simulink model "sm_car_"  (R2026b)
settings: Solver=ode23t  StopTime=100  MaxStep=0.4  AbsTol=1e-3  EnableMultiTasking=on
PreLoadFcn:
  | % Due to usability issue in Repeating Sequence block
  | warning('off','Simulink:Masking:Invalid');
  | 
  | % Eliminate unnecessary warnings in inactive variants
  | % Warnings generated only if you click through inactive variant
  | warning('off','MATLAB:nonExistentField');
  | warning('off','Simulink:Parameters:BlkParamUndefined');
PostLoadFcn:
  | set_param([bdroot '/Vehicle'],'popup_trailer','Off')
  | warning('off','sm:sli:setup:compile:LocalSolverNotSupported')
  | %sm_car_config_maneuver(bdroot,'WOT Braking');
  | sm_car_config_vehicle(bdroot,'false');
  | sm_car_config_logging(bdroot);
InitFcn:
  | sm_car_config_camera;
  | Vehicle = sm_car_vehcfg_checkConfig(Vehicle);
  | sm_car_check_tire_model(bdroot);
StartFcn:
  | tic;
StopFcn:
  | Elapsed_Sim_Time = toc;
  | % disp(['Elapsed Sim Time = ' num2str(Elapsed_Sim_Time)]);
undefined symbols (not defined in the file or in its folder): acc_theta, accel_ramp_rate, Axle1D, AxleIn, Camera, Control, Driver, Init, Maneuver, Pedal, Scene, ShaftL1, ShaftL2, ShaftR1, ShaftR2, Visual, X, xy_data_car_side, Y, Z
libraries: sm_lib x290, fl_lib x171, nesl_utility x144, simulink x60, simulink_extras x14, sdl_lib x14, SimscapeFluids_lib x7, Damper_Element x4, Tire_1x2x x4, ee_lib x3, Scene_Utilities x3, sharedTrackingLibrary x2
(part 17 of 22)

== system sm_car_/World/Scene/CRG Hockenheim F/Finish Line/R5 ==
  Square LL : sm_lib/Body Elements/Brick Solid  BrickDimensions=square_lwh  BrickDimensionsUnits=m  ExportEntireGeometry=off  InertiaType=CalculateFromGeometry  BasedOnType=Density  Density=1000  DensityUnits=kg/m^3  Mass=1  MassUnits=kg  CenterOfMass=[0 0 0]  CenterOfMassUnits=m  MomentsOfInertia=[1 1 1]  MomentsOfInertiaUnits=kg*m^2  ProductsOfInertia=[0 0 0]  ProductsOfInertiaUnits=kg*m^2  GraphicType=FromGeometry  MarkerShape=Sphere  MarkerSize=10  GraphicVisPropType=SimpleVisualProperties  GraphicDiffuseColor=[0.0 0.0 0.0]  GraphicOpacity=1.0  GraphicSpecularColor=[0.5 0.5 0.5 1.0]  GraphicAmbientColor=[0.15 0.15 0.15 1.0]  GraphicEmissiveColor=[0.0 0.0 0.0 1.0]  GraphicShininess=75  DoExposeReferenceFrame=off  SerializedFrames=<Frames><Frame><Id>Frame1</Id><Value><Name>BL</Name><Origin><Source>GeometricFeature</Source><FeatureName>+y -z curve</FeatureName></Origin><PrimaryAxis><DefinedDirection>+Z</DefinedDirection><Source>ReferenceFrame</Source><SourceDirection>+Z</SourceDirection><FeatureName></FeatureName></PrimaryAxis><SecondaryAxis><DefinedDirection>+X</DefinedDirection><Source>ReferenceFrame</Source><SourceDirection>+X</SourceDirection><FeatureName></FeatureName></SecondaryAxis></Value></Frame><Frame><Id>Frame2</Id><Value><Name>TL</Name><Origin><Source>GeometricFeature</Source><FeatureName>+x +y +z point</FeatureName></Origin><PrimaryAxis><DefinedDirection>+Z</DefinedDirection><Source>ReferenceFrame</Source><SourceDirection>+Z</SourceDirection><FeatureName></FeatureName></PrimaryAxis><SecondaryAxis><DefinedDirection>+X</DefinedDirection><Source>ReferenceFrame</Source><SourceDirection>+X</SourceDirection><FeatureName></FeatureName></SecondaryAxis></Value></Frame><Frame><Id>Frame3</Id><Value><Name>BR</Name><Origin><Source>GeometricFeature</Source><FeatureName>-y -z curve</FeatureName></Origin><PrimaryAxis><DefinedDirection>+Z</DefinedDirection><Source>ReferenceFrame</Source><SourceDirection>+Z</SourceDirection><FeatureName></FeatureName></PrimaryAxis><SecondaryAxis><DefinedDirection>+X</DefinedDirection><Source>ReferenceFrame</Source><SourceDirection>+X</SourceDirection><FeatureName></FeatureName></SecondaryAxis></Value></Frame></Frames>
  Square LR : sm_lib/Body Elements/Brick Solid  BrickDimensions=square_lwh  BrickDimensionsUnits=m  ExportEntireGeometry=off  InertiaType=CalculateFromGeometry  BasedOnType=Density  Density=1000  DensityUnits=kg/m^3  Mass=1  MassUnits=kg  CenterOfMass=[0 0 0]  CenterOfMassUnits=m  MomentsOfInertia=[1 1 1]  MomentsOfInertiaUnits=kg*m^2  ProductsOfInertia=[0 0 0]  ProductsOfInertiaUnits=kg*m^2  GraphicType=FromGeometry  MarkerShape=Sphere  MarkerSize=10  GraphicVisPropType=SimpleVisualProperties  GraphicDiffuseColor=[1.0 1.0 1.0]  GraphicOpacity=1.0  GraphicSpecularColor=[0.5 0.5 0.5 1.0]  GraphicAmbientColor=[0.15 0.15 0.15 1.0]  GraphicEmissiveColor=[0.0 0.0 0.0 1.0]  GraphicShininess=75  DoExposeReferenceFrame=off  SerializedFrames=<Frames><Frame><Id>Frame1</Id><Value><Name>BL</Name><Origin><Source>GeometricFeature</Source><FeatureName>+y -z curve</FeatureName></Origin><PrimaryAxis><DefinedDirection>+Z</DefinedDirection><Source>ReferenceFrame</Source><SourceDirection>+Z</SourceDirection><FeatureName></FeatureName></PrimaryAxis><SecondaryAxis><DefinedDirection>+X</DefinedDirection><Source>ReferenceFrame</Source><SourceDirection>+X</SourceDirection><FeatureName></FeatureName></SecondaryAxis></Value></Frame><Frame><Id>Frame2</Id><Value><Name>TL</Name><Origin><Source>GeometricFeature</Source><FeatureName>+x +y +z point</FeatureName></Origin><PrimaryAxis><DefinedDirection>+Z</DefinedDirection><Source>ReferenceFrame</Source><SourceDirection>+Z</SourceDirection><FeatureName></FeatureName></PrimaryAxis><SecondaryAxis><DefinedDirection>+X</DefinedDirection><Source>ReferenceFrame</Source><SourceDirection>+X</SourceDirection><FeatureName></FeatureName></SecondaryAxis></Value></Frame><Frame><Id>Frame3</Id><Value><Name>BR</Name><Origin><Source>GeometricFeature</Source><FeatureName>-y -z curve</FeatureName></Origin><PrimaryAxis><DefinedDirection>+Z</DefinedDirection><Source>ReferenceFrame</Source><SourceDirection>+Z</SourceDirection><FeatureName></FeatureName></PrimaryAxis><SecondaryAxis><DefinedDirection>+X</DefinedDirection><Source>ReferenceFrame</Source><SourceDirection>+X</SourceDirection><FeatureName></FeatureName></SecondaryAxis></Value></Frame></Frames>
  Square UL : sm_lib/Body Elements/Brick Solid  BrickDimensions=square_lwh  BrickDimensionsUnits=m  ExportEntireGeometry=off  InertiaType=CalculateFromGeometry  BasedOnType=Density  Density=1000  DensityUnits=kg/m^3  Mass=1  MassUnits=kg  CenterOfMass=[0 0 0]  CenterOfMassUnits=m  MomentsOfInertia=[1 1 1]  MomentsOfInertiaUnits=kg*m^2  ProductsOfInertia=[0 0 0]  ProductsOfInertiaUnits=kg*m^2  GraphicType=FromGeometry  MarkerShape=Sphere  MarkerSize=10  GraphicVisPropType=SimpleVisualProperties  GraphicDiffuseColor=[1.0 1.0 1.0]  GraphicOpacity=1.0  GraphicSpecularColor=[0.5 0.5 0.5 1.0]  GraphicAmbientColor=[0.15 0.15 0.15 1.0]  GraphicEmissiveColor=[0.0 0.0 0.0 1.0]  GraphicShininess=75  DoExposeReferenceFrame=off  SerializedFrames=<Frames><Frame><Id>Frame1</Id><Value><Name>BL</Name><Origin><Source>GeometricFeature</Source><FeatureName>+y -z curve</FeatureName></Origin><PrimaryAxis><DefinedDirection>+Z</DefinedDirection><Source>ReferenceFrame</Source><SourceDirection>+Z</SourceDirection><FeatureName></FeatureName></PrimaryAxis><SecondaryAxis><DefinedDirection>+X</DefinedDirection><Source>ReferenceFrame</Source><SourceDirection>+X</SourceDirection><FeatureName></FeatureName></SecondaryAxis></Value></Frame><Frame><Id>Frame2</Id><Value><Name>TL</Name><Origin><Source>GeometricFeature</Source><FeatureName>+x +y +z point</FeatureName></Origin><PrimaryAxis><DefinedDirection>+Z</DefinedDirection><Source>ReferenceFrame</Source><SourceDirection>+Z</SourceDirection><FeatureName></FeatureName></PrimaryAxis><SecondaryAxis><DefinedDirection>+X</DefinedDirection><Source>ReferenceFrame</Source><SourceDirection>+X</SourceDirection><FeatureName></FeatureName></SecondaryAxis></Value></Frame><Frame><Id>Frame3</Id><Value><Name>BR</Name><Origin><Source>GeometricFeature</Source><FeatureName>-y -z curve</FeatureName></Origin><PrimaryAxis><DefinedDirection>+Z</DefinedDirection><Source>ReferenceFrame</Source><SourceDirection>+Z</SourceDirection><FeatureName></FeatureName></PrimaryAxis><SecondaryAxis><DefinedDirection>+X</DefinedDirection><Source>ReferenceFrame</Source><SourceDirection>+X</SourceDirection><FeatureName></FeatureName></SecondaryAxis></Value></Frame></Frames>
  Square UR : sm_lib/Body Elements/Brick Solid  BrickDimensions=square_lwh  BrickDimensionsUnits=m  ExportEntireGeometry=off  InertiaType=CalculateFromGeometry  BasedOnType=Density  Density=1000  DensityUnits=kg/m^3  Mass=1  MassUnits=kg  CenterOfMass=[0 0 0]  CenterOfMassUnits=m  MomentsOfInertia=[1 1 1]  MomentsOfInertiaUnits=kg*m^2  ProductsOfInertia=[0 0 0]  ProductsOfInertiaUnits=kg*m^2  GraphicType=FromGeometry  MarkerShape=Sphere  MarkerSize=10  GraphicVisPropType=SimpleVisualProperties  GraphicDiffuseColor=[0.0 0.0 0.0]  GraphicOpacity=1.0  GraphicSpecularColor=[0.5 0.5 0.5 1.0]  GraphicAmbientColor=[0.15 0.15 0.15 1.0]  GraphicEmissiveColor=[0.0 0.0 0.0 1.0]  GraphicShininess=75  DoExposeReferenceFrame=off  SerializedFrames=<Frames><Frame><Id>Frame1</Id><Value><Name>BL</Name><Origin><Source>GeometricFeature</Source><FeatureName>+y -z curve</FeatureName></Origin><PrimaryAxis><DefinedDirection>+Z</DefinedDirection><Source>ReferenceFrame</Source><SourceDirection>+Z</SourceDirection><FeatureName></FeatureName></PrimaryAxis><SecondaryAxis><DefinedDirection>+X</DefinedDirection><Source>ReferenceFrame</Source><SourceDirection>+X</SourceDirection><FeatureName></FeatureName></SecondaryAxis></Value></Frame><Frame><Id>Frame2</Id><Value><Name>TL</Name><Origin><Source>GeometricFeature</Source><FeatureName>+x +y +z point</FeatureName></Origin><PrimaryAxis><DefinedDirection>+Z</DefinedDirection><Source>ReferenceFrame</Source><SourceDirection>+Z</SourceDirection><FeatureName></FeatureName></PrimaryAxis><SecondaryAxis><DefinedDirection>+X</DefinedDirection><Source>ReferenceFrame</Source><SourceDirection>+X</SourceDirection><FeatureName></FeatureName></SecondaryAxis></Value></Frame><Frame><Id>Frame3</Id><Value><Name>BR</Name><Origin><Source>GeometricFeature</Source><FeatureName>-y -z curve</FeatureName></Origin><PrimaryAxis><DefinedDirection>+Z</DefinedDirection><Source>ReferenceFrame</Source><SourceDirection>+Z</SourceDirection><FeatureName></FeatureName></PrimaryAxis><SecondaryAxis><DefinedDirection>+X</DefinedDirection><Source>ReferenceFrame</Source><SourceDirection>+X</SourceDirection><FeatureName></FeatureName></SecondaryAxis></Value></Frame></Frames>
  BL : PMIOPort  Side=Left
  BR : PMIOPort  Port=2  Side=Right
  connections:
  Square LR/LConn1 -- Square LL/LConn2
  Square LL/LConn1 -- BL/RConn1
  Square UL/LConn1 -- Square LL/RConn1
  Square UR/LConn1 -- Square LR/RConn1
  BR/RConn1 -- Square LR/LConn2

== system sm_car_/World/Scene/Plane Grid/Grid/Mesh Lines x ==
  Solid : sm_lib/Body Elements/Extruded Solid  ExtrusionType=General  PolygonNumSides=3  PolygonOuterRadius=1  PolygonOuterRadiusUnits=m  ExportEntireGeometry=off  ExtrusionCrossSection=mesh_xsec  ExtrusionCrossSectionUnits=m  ExportConvexHullGeometry=off  ExtrusionLength=mesh_thickness  ExtrusionLengthUnits=m  InertiaType=CalculateFromGeometry  BasedOnType=Density  Density=mesh_rho  DensityUnits=kg/(m^3)  Mass=1  MassUnits=kg  CenterOfMass=[0 0 0]  CenterOfMassUnits=m  MomentsOfInertia=[1 1 1]  MomentsOfInertiaUnits=kg*m^2  ProductsOfInertia=[0 0 0]  ProductsOfInertiaUnits=kg*m^2  GraphicType=FromGeometry  MarkerShape=Sphere  MarkerSize=10  GraphicVisPropType=SimpleVisualProperties  GraphicDiffuseColor=mesh_color  GraphicOpacity=mesh_opc  GraphicSpecularColor=[0.5 0.5 0.5 1.0]  GraphicAmbientColor=[0.15 0.15 0.15 1.0]  GraphicEmissiveColor=[0.0 0.0 0.0 1.0]  GraphicShininess=75  DoExposeReferenceFrame=on  SerializedFrames=<Frames/>
  Transform Bottom : sm_lib/Frames and Transforms/Rigid Transform  RotationMethod=None  FollAlignAxisA=+X  BaseAlignAxisA=+Y  FollAlignAxisB=+Y  BaseAlignAxisB=+Z  RotationStandardAxis=+Z  RotationAngle=0.0  RotationAngleUnits=deg  RotationArbitraryAxis=[0 0 1]  RotationSequenceAxes=FollowerAxes  RotationSequence=XYX  RotationSequenceAngles=[0 0 0]  RotationSequenceAnglesUnits=deg  RotationMatrix=[1 0 0; 0 1 0; 0 0 1]  Quaternion=[1 0 0 0]  TranslationMethod=StandardAxis  TranslationCartesianOffset=[0 0 0]  TranslationCartesianOffsetUnits=m  TranslationStandardAxis=-Z  TranslationStandardOffset=mesh_thickness/2  TranslationStandardOffsetUnits=m  TranslationROffset=0  TranslationROffsetUnits=m  TranslationThetaOffset=0  TranslationThetaOffsetUnits=deg  TranslationZOffset=0  TranslationZOffsetUnits=m
  Transform Top : sm_lib/Frames and Transforms/Rigid Transform  RotationMethod=None  FollAlignAxisA=+X  BaseAlignAxisA=+Y  FollAlignAxisB=+Y  BaseAlignAxisB=+Z  RotationStandardAxis=+Z  RotationAngle=0.0  RotationAngleUnits=deg  RotationArbitraryAxis=[0 0 1]  RotationSequenceAxes=FollowerAxes  RotationSequence=XYX  RotationSequenceAngles=[0 0 0]  RotationSequenceAnglesUnits=deg  RotationMatrix=[1 0 0; 0 1 0; 0 0 1]  Quaternion=[1 0 0 0]  TranslationMethod=StandardAxis  TranslationCartesianOffset=[0 0 0]  TranslationCartesianOffsetUnits=m  TranslationStandardAxis=+Z  TranslationStandardOffset=mesh_thickness/2  TranslationStandardOffsetUnits=m  TranslationROffset=0  TranslationROffsetUnits=m  TranslationThetaOffset=0  TranslationThetaOffsetUnits=deg  TranslationZOffset=0  TranslationZOffsetUnits=m
  F : PMIOPort  Side=Right
  R : PMIOPort  Port=2  Side=Left
  B : PMIOPort  Port=3  Side=Right
  connections:
  F/RConn1 -- Transform Top/RConn1
  B/RConn1 -- Transform Bottom/RConn1
  R/RConn1 -- Transform Top/LConn1 -- Transform Bottom/LConn1 -- Solid/RConn1

== system sm_car_/World/Scene/Plane Grid/Grid/Mesh Lines y  ==
  Solid : sm_lib/Body Elements/Extruded Solid  ExtrusionType=General  PolygonNumSides=3  PolygonOuterRadius=1  PolygonOuterRadiusUnits=m  ExportEntireGeometry=off  ExtrusionCrossSection=mesh_xsec  ExtrusionCrossSectionUnits=m  ExportConvexHullGeometry=off  ExtrusionLength=mesh_thickness  ExtrusionLengthUnits=m  InertiaType=CalculateFromGeometry  BasedOnType=Density  Density=mesh_rho  DensityUnits=kg/(m^3)  Mass=1  MassUnits=kg  CenterOfMass=[0 0 0]  CenterOfMassUnits=m  MomentsOfInertia=[1 1 1]  MomentsOfInertiaUnits=kg*m^2  ProductsOfInertia=[0 0 0]  ProductsOfInertiaUnits=kg*m^2  GraphicType=FromGeometry  MarkerShape=Sphere  MarkerSize=10  GraphicVisPropType=SimpleVisualProperties  GraphicDiffuseColor=mesh_color  GraphicOpacity=mesh_opc  GraphicSpecularColor=[0.5 0.5 0.5 1.0]  GraphicAmbientColor=[0.15 0.15 0.15 1.0]  GraphicEmissiveColor=[0.0 0.0 0.0 1.0]  GraphicShininess=75  DoExposeReferenceFrame=on  SerializedFrames=<Frames/>
  Transform Bottom : sm_lib/Frames and Transforms/Rigid Transform  RotationMethod=None  FollAlignAxisA=+X  BaseAlignAxisA=+Y  FollAlignAxisB=+Y  BaseAlignAxisB=+Z  RotationStandardAxis=+Z  RotationAngle=0.0  RotationAngleUnits=deg  RotationArbitraryAxis=[0 0 1]  RotationSequenceAxes=FollowerAxes  RotationSequence=XYX  RotationSequenceAngles=[0 0 0]  RotationSequenceAnglesUnits=deg  RotationMatrix=[1 0 0; 0 1 0; 0 0 1]  Quaternion=[1 0 0 0]  TranslationMethod=StandardAxis  TranslationCartesianOffset=[0 0 0]  TranslationCartesianOffsetUnits=m  TranslationStandardAxis=-Z  TranslationStandardOffset=mesh_thickness/2  TranslationStandardOffsetUnits=m  TranslationROffset=0  TranslationROffsetUnits=m  TranslationThetaOffset=0  TranslationThetaOffsetUnits=deg  TranslationZOffset=0  TranslationZOffsetUnits=m
  Transform Top : sm_lib/Frames and Transforms/Rigid Transform  RotationMethod=None  FollAlignAxisA=+X  BaseAlignAxisA=+Y  FollAlignAxisB=+Y  BaseAlignAxisB=+Z  RotationStandardAxis=+Z  RotationAngle=0.0  RotationAngleUnits=deg  RotationArbitraryAxis=[0 0 1]  RotationSequenceAxes=FollowerAxes  RotationSequence=XYX  RotationSequenceAngles=[0 0 0]  RotationSequenceAnglesUnits=deg  RotationMatrix=[1 0 0; 0 1 0; 0 0 1]  Quaternion=[1 0 0 0]  TranslationMethod=StandardAxis  TranslationCartesianOffset=[0 0 0]  TranslationCartesianOffsetUnits=m  TranslationStandardAxis=+Z  TranslationStandardOffset=mesh_thickness/2  TranslationStandardOffsetUnits=m  TranslationROffset=0  TranslationROffsetUnits=m  TranslationThetaOffset=0  TranslationThetaOffsetUnits=deg  TranslationZOffset=0  TranslationZOffsetUnits=m
  F : PMIOPort  Side=Right
  R : PMIOPort  Port=2  Side=Left
  B : PMIOPort  Port=3  Side=Right
  connections:
  F/RConn1 -- Transform Top/RConn1
  B/RConn1 -- Transform Bottom/RConn1
  R/RConn1 -- Transform Top/LConn1 -- Transform Bottom/LConn1 -- Solid/RConn1

== system sm_car_/Controller/TrqVec 4Motor/Brake Control/ABS/Sensor/missing tooth ==
  <omega> : Inport
  <qxyz> : Inport  Port=2
  Constant : Constant  Value=2*pi
  Constant1 : Constant  Value=0.5
  Constant2 : Constant
  Product : Product
  Rem : Math  Operator=rem  SignedPower=on
  Scope : Scope  NumInputPorts=5
      settings: ActiveDisplayYMinimum=-41.32335  ActiveDisplayYMaximum=259.55855  DataLoggingVariableName=ScopeData2
  Selector : Selector  InputPortWidth=3  IndexOptions=Index vector (dialog)  Indices=[2]  OutputSizes=1  RuntimeRangeChecks=off
  Subsystem : Subsystem  mask{int_limit_upper=25/48*2*pi, int_limit_lower=22/48*2*pi}
      mask prompts: int_limit_upper "Upper Limit"; int_limit_lower "Lower Limit"
      mask TypeOptions int_limit_upper: Upper Limit/Value
      mask TypeOptions int_limit_lower: Lower Limit/Value
  Switch : Switch  Criteria=u2 > Threshold  Threshold=0.5  SaturateOnIntegerOverflow=off  InputSameDT=off
  Out1 : Outport  VectorParamsAs1DForOutWhenUnconnected=off
  wires:
  <qxyz>/1 -> Scope/1, Selector/1
  Constant/1 -> Rem/2
  Rem/1 -> Scope/3, Subsystem/1(u)
  Selector/1 -> Scope/2, Rem/1
  Subsystem/1(y) -> Scope/4, Switch/2
  Switch/1 -> Scope/5, Product/2
  Constant1/1 -> Switch/1
  Constant2/1 -> Switch/3
  <omega>/1 -> Product/1
  Product/1 -> Out1/1

== system sm_car_/Controller/TrqVec 4Motor/Brake Control/ABS/Valve Control L1/Categorize Surface ==
  Mod State : Inport
  Apply Valve : Inport  Port=2
  Compare To Constant : simulink/Logic and Bit Operations/Compare To Constant  relop=<  const=4  OutDataTypeStr=boolean
  Compare To Constant1 : simulink/Logic and Bit Operations/Compare To Constant  relop===  const=2  OutDataTypeStr=boolean
  Count Apply Pulses : Subsystem  TreatAsAtomicUnit=on
  Terminator : Terminator
  Total Apply Pulses This Cycle : Subsystem  TreatAsAtomicUnit=on
  wires:
  Compare To Constant/1 -> Terminator/1  "Low Mu"
  Total Apply Pulses This Cycle/1(Total Pulses) -> Compare To Constant/1
  Compare To Constant1/1 -> Count Apply Pulses/1(In1)
  Mod State/1 -> Compare To Constant1/1, Total Apply Pulses This Cycle/Trigger  "Transition to Release"
  Apply Valve/1 -> Count Apply Pulses/Trigger
  Count Apply Pulses/1(Apply Pulses) -> Total Apply Pulses This Cycle/1(In1)

== system sm_car_/Controller/TrqVec 4Motor/Brake Control/ABS/Valve Control L1/Code to Valves ==
  note: Release
  note: Hold
  note: Apply
  C : Inport
  Constant : Constant  Value=[0 0]
  Constant1 : Constant  Value=[0 1]
  Constant2 : Constant  Value=[1 0]
  Multiport Switch : MultiPortSwitch  DataPortOrder=Zero-based contiguous  zeroidx=on  SaturateOnIntegerOverflow=off  InputSameDT=off
  V : Outport  VectorParamsAs1DForOutWhenUnconnected=off
  wires:
  Multiport Switch/1 -> V/1
  C/1 -> Multiport Switch/1
  Constant2/1 -> Multiport Switch/4
  Constant1/1 -> Multiport Switch/3
  Constant/1 -> Multiport Switch/2

== system sm_car_/Controller/TrqVec 4Motor/Brake Control/ABS/Valve Control L1/Subsystem ==
  OnT : Inport
  Constant : Constant  Value=0
  Constant1 : Constant
  Demux : Demux  Outputs=9
  Multiport Switch : MultiPortSwitch  DataPortOrder=Zero-based contiguous  Inputs=11  zeroidx=on  SaturateOnIntegerOverflow=off  InputSameDT=off
  Pulse Generator : DiscretePulseGenerator  PulseType=Time based  Period=0.01  PulseWidth=[1 2 3 4 5 6 7 8 9]*10
  vSig : Outport  VectorParamsAs1DForOutWhenUnconnected=off
  wires:
  Multiport Switch/1 -> vSig/1
  Demux/9 -> Multiport Switch/11
  Demux/8 -> Multiport Switch/10
  Demux/7 -> Multiport Switch/9
  Demux/6 -> Multiport Switch/8
  Demux/5 -> Multiport Switch/7
  Demux/4 -> Multiport Switch/6
  Demux/3 -> Multiport Switch/5
  Demux/2 -> Multiport Switch/4
  Demux/1 -> Multiport Switch/3
  OnT/1 -> Multiport Switch/1
  Constant1/1 -> Multiport Switch/12
  Constant/1 -> Multiport Switch/2
  Pulse Generator/1 -> Demux/1

== system sm_car_/Controller/TrqVec 4Motor/Brake Control/ABS/Valve Control L1/Subsystem1 ==
  OnT : Inport
  Constant : Constant  Value=0
  Constant1 : Constant
  Demux : Demux  Outputs=9
  Multiport Switch : MultiPortSwitch  DataPortOrder=Zero-based contiguous  Inputs=11  zeroidx=on  SaturateOnIntegerOverflow=off  InputSameDT=off
  Pulse Generator : DiscretePulseGenerator  PulseType=Time based  Period=0.01  PulseWidth=[1 2 3 4 5 6 7 8 9]*10
  vSig : Outport  VectorParamsAs1DForOutWhenUnconnected=off
  wires:
  Pulse Generator/1 -> Demux/1
  Constant/1 -> Multiport Switch/2
  Constant1/1 -> Multiport Switch/12
  OnT/1 -> Multiport Switch/1
  Demux/1 -> Multiport Switch/3
  Demux/2 -> Multiport Switch/4
  Demux/3 -> Multiport Switch/5
  Demux/4 -> Multiport Switch/6
  Demux/5 -> Multiport Switch/7
  Demux/6 -> Multiport Switch/8
  Demux/7 -> Multiport Switch/9
  Demux/8 -> Multiport Switch/10
  Demux/9 -> Multiport Switch/11
  Multiport Switch/1 -> vSig/1

== system sm_car_/Controller/TrqVec 4Motor/Brake Control/ABS/Valve Control L2/Categorize Surface ==
  Mod State : Inport
  Apply Valve : Inport  Port=2
  Compare To Constant : simulink/Logic and Bit Operations/Compare To Constant  relop=<  const=4  OutDataTypeStr=boolean
  Compare To Constant1 : simulink/Logic and Bit Operations/Compare To Constant  relop===  const=2  OutDataTypeStr=boolean
  Count Apply Pulses : Subsystem  TreatAsAtomicUnit=on
  Terminator : Terminator
  Total Apply Pulses This Cycle : Subsystem  TreatAsAtomicUnit=on
  wires:
  Compare To Constant/1 -> Terminator/1  "Low Mu"
  Total Apply Pulses This Cycle/1(Total Pulses) -> Compare To Constant/1
  Compare To Constant1/1 -> Count Apply Pulses/1(In1)
  Mod State/1 -> Compare To Constant1/1, Total Apply Pulses This Cycle/Trigger  "Transition to Release"
  Apply Valve/1 -> Count Apply Pulses/Trigger
  Count Apply Pulses/1(Apply Pulses) -> Total Apply Pulses This Cycle/1(In1)

== system sm_car_/Controller/TrqVec 4Motor/Brake Control/ABS/Valve Control L2/Code to Valves ==
  note: Release
  note: Hold
  note: Apply
  C : Inport
  Constant : Constant  Value=[0 0]
  Constant1 : Constant  Value=[0 1]
  Constant2 : Constant  Value=[1 0]
  Multiport Switch : MultiPortSwitch  DataPortOrder=Zero-based contiguous  zeroidx=on  SaturateOnIntegerOverflow=off  InputSameDT=off
  V : Outport  VectorParamsAs1DForOutWhenUnconnected=off
  wires:
  Multiport Switch/1 -> V/1
  C/1 -> Multiport Switch/1
  Constant2/1 -> Multiport Switch/4
  Constant1/1 -> Multiport Switch/3
  Constant/1 -> Multiport Switch/2

== system sm_car_/Controller/TrqVec 4Motor/Brake Control/ABS/Valve Control L2/Subsystem ==
  OnT : Inport
  Constant : Constant  Value=0
  Constant1 : Constant
  Demux : Demux  Outputs=9
  Multiport Switch : MultiPortSwitch  DataPortOrder=Zero-based contiguous  Inputs=11  zeroidx=on  SaturateOnIntegerOverflow=off  InputSameDT=off
  Pulse Generator : DiscretePulseGenerator  PulseType=Time based  Period=0.01  PulseWidth=[1 2 3 4 5 6 7 8 9]*10
  vSig : Outport  VectorParamsAs1DForOutWhenUnconnected=off
  wires:
  Multiport Switch/1 -> vSig/1
  Demux/9 -> Multiport Switch/11
  Demux/8 -> Multiport Switch/10
  Demux/7 -> Multiport Switch/9
  Demux/6 -> Multiport Switch/8
  Demux/5 -> Multiport Switch/7
  Demux/4 -> Multiport Switch/6
  Demux/3 -> Multiport Switch/5
  Demux/2 -> Multiport Switch/4
  Demux/1 -> Multiport Switch/3
  OnT/1 -> Multiport Switch/1
  Constant1/1 -> Multiport Switch/12
  Constant/1 -> Multiport Switch/2
  Pulse Generator/1 -> Demux/1

== system sm_car_/Controller/TrqVec 4Motor/Brake Control/ABS/Valve Control L2/Subsystem1 ==
  OnT : Inport
  Constant : Constant  Value=0
  Constant1 : Constant
  Demux : Demux  Outputs=9
  Multiport Switch : MultiPortSwitch  DataPortOrder=Zero-based contiguous  Inputs=11  zeroidx=on  SaturateOnIntegerOverflow=off  InputSameDT=off
  Pulse Generator : DiscretePulseGenerator  PulseType=Time based  Period=0.01  PulseWidth=[1 2 3 4 5 6 7 8 9]*10
  vSig : Outport  VectorParamsAs1DForOutWhenUnconnected=off
  wires:
  Pulse Generator/1 -> Demux/1
  Constant/1 -> Multiport Switch/2
  Constant1/1 -> Multiport Switch/12
  OnT/1 -> Multiport Switch/1
  Demux/1 -> Multiport Switch/3
  Demux/2 -> Multiport Switch/4
  Demux/3 -> Multiport Switch/5
  Demux/4 -> Multiport Switch/6
  Demux/5 -> Multiport Switch/7
  Demux/6 -> Multiport Switch/8
  Demux/7 -> Multiport Switch/9
  Demux/8 -> Multiport Switch/10
  Demux/9 -> Multiport Switch/11
  Multiport Switch/1 -> vSig/1

== system sm_car_/Controller/TrqVec 4Motor/Brake Control/ABS/Valve Control R1/Categorize Surface ==
  Mod State : Inport
  Apply Valve : Inport  Port=2
  Compare To Constant : simulink/Logic and Bit Operations/Compare To Constant  relop=<  const=4  OutDataTypeStr=boolean
  Compare To Constant1 : simulink/Logic and Bit Operations/Compare To Constant  relop===  const=2  OutDataTypeStr=boolean
  Count Apply Pulses : Subsystem  TreatAsAtomicUnit=on
  Terminator : Terminator
  Total Apply Pulses This Cycle : Subsystem  TreatAsAtomicUnit=on
  wires:
  Compare To Constant/1 -> Terminator/1  "Low Mu"
  Total Apply Pulses This Cycle/1(Total Pulses) -> Compare To Constant/1
  Compare To Constant1/1 -> Count Apply Pulses/1(In1)
  Mod State/1 -> Compare To Constant1/1, Total Apply Pulses This Cycle/Trigger  "Transition to Release"
  Apply Valve/1 -> Count Apply Pulses/Trigger
  Count Apply Pulses/1(Apply Pulses) -> Total Apply Pulses This Cycle/1(In1)

== system sm_car_/Controller/TrqVec 4Motor/Brake Control/ABS/Valve Control R1/Code to Valves ==
  note: Release
  note: Hold
  note: Apply
  C : Inport
  Constant : Constant  Value=[0 0]
  Constant1 : Constant  Value=[0 1]
  Constant2 : Constant  Value=[1 0]
  Multiport Switch : MultiPortSwitch  DataPortOrder=Zero-based contiguous  zeroidx=on  SaturateOnIntegerOverflow=off  InputSameDT=off
  V : Outport  VectorParamsAs1DForOutWhenUnconnected=off
  wires:
  Multiport Switch/1 -> V/1
  C/1 -> Multiport Switch/1
  Constant2/1 -> Multiport Switch/4
  Constant1/1 -> Multiport Switch/3
  Constant/1 -> Multiport Switch/2

== system sm_car_/Controller/TrqVec 4Motor/Brake Control/ABS/Valve Control R1/Subsystem ==
  OnT : Inport
  Constant : Constant  Value=0
  Constant1 : Constant
  Demux : Demux  Outputs=9
  Multiport Switch : MultiPortSwitch  DataPortOrder=Zero-based contiguous  Inputs=11  zeroidx=on  SaturateOnIntegerOverflow=off  InputSameDT=off
  Pulse Generator : DiscretePulseGenerator  PulseType=Time based  Period=0.01  PulseWidth=[1 2 3 4 5 6 7 8 9]*10
  vSig : Outport  VectorParamsAs1DForOutWhenUnconnected=off
  wires:
  Multiport Switch/1 -> vSig/1
  Demux/9 -> Multiport Switch/11
  Demux/8 -> Multiport Switch/10
  Demux/7 -> Multiport Switch/9
  Demux/6 -> Multiport Switch/8
  Demux/5 -> Multiport Switch/7
  Demux/4 -> Multiport Switch/6
  Demux/3 -> Multiport Switch/5
  Demux/2 -> Multiport Switch/4
  Demux/1 -> Multiport Switch/3
  OnT/1 -> Multiport Switch/1
  Constant1/1 -> Multiport Switch/12
  Constant/1 -> Multiport Switch/2
  Pulse Generator/1 -> Demux/1

== system sm_car_/Controller/TrqVec 4Motor/Brake Control/ABS/Valve Control R1/Subsystem1 ==
  OnT : Inport
  Constant : Constant  Value=0
  Constant1 : Constant
  Demux : Demux  Outputs=9
  Multiport Switch : MultiPortSwitch  DataPortOrder=Zero-based contiguous  Inputs=11  zeroidx=on  SaturateOnIntegerOverflow=off  InputSameDT=off
  Pulse Generator : DiscretePulseGenerator  PulseType=Time based  Period=0.01  PulseWidth=[1 2 3 4 5 6 7 8 9]*10
  vSig : Outport  VectorParamsAs1DForOutWhenUnconnected=off
  wires:
  Pulse Generator/1 -> Demux/1
  Constant/1 -> Multiport Switch/2
  Constant1/1 -> Multiport Switch/12
  OnT/1 -> Multiport Switch/1
  Demux/1 -> Multiport Switch/3
  Demux/2 -> Multiport Switch/4
  Demux/3 -> Multiport Switch/5
  Demux/4 -> Multiport Switch/6
  Demux/5 -> Multiport Switch/7
  Demux/6 -> Multiport Switch/8
  Demux/7 -> Multiport Switch/9
  Demux/8 -> Multiport Switch/10
  Demux/9 -> Multiport Switch/11
  Multiport Switch/1 -> vSig/1

== system sm_car_/Controller/TrqVec 4Motor/Brake Control/ABS/Valve Control R2/Categorize Surface ==
  Mod State : Inport
  Apply Valve : Inport  Port=2
  Compare To Constant : simulink/Logic and Bit Operations/Compare To Constant  relop=<  const=4  OutDataTypeStr=boolean
  Compare To Constant1 : simulink/Logic and Bit Operations/Compare To Constant  relop===  const=2  OutDataTypeStr=boolean
  Count Apply Pulses : Subsystem  TreatAsAtomicUnit=on
  Terminator : Terminator
  Total Apply Pulses This Cycle : Subsystem  TreatAsAtomicUnit=on
  wires:
  Compare To Constant/1 -> Terminator/1  "Low Mu"
  Total Apply Pulses This Cycle/1(Total Pulses) -> Compare To Constant/1
  Compare To Constant1/1 -> Count Apply Pulses/1(In1)
  Mod State/1 -> Compare To Constant1/1, Total Apply Pulses This Cycle/Trigger  "Transition to Release"
  Apply Valve/1 -> Count Apply Pulses/Trigger
  Count Apply Pulses/1(Apply Pulses) -> Total Apply Pulses This Cycle/1(In1)

== system sm_car_/Controller/TrqVec 4Motor/Brake Control/ABS/Valve Control R2/Code to Valves ==
  note: Release
  note: Hold
  note: Apply
  C : Inport
  Constant : Constant  Value=[0 0]
  Constant1 : Constant  Value=[0 1]
  Constant2 : Constant  Value=[1 0]
  Multiport Switch : MultiPortSwitch  DataPortOrder=Zero-based contiguous  zeroidx=on  SaturateOnIntegerOverflow=off  InputSameDT=off
  V : Outport  VectorParamsAs1DForOutWhenUnconnected=off
  wires:
  Multiport Switch/1 -> V/1
  C/1 -> Multiport Switch/1
  Constant2/1 -> Multiport Switch/4
  Constant1/1 -> Multiport Switch/3
  Constant/1 -> Multiport Switch/2

== system sm_car_/Controller/TrqVec 4Motor/Brake Control/ABS/Valve Control R2/Subsystem ==
  OnT : Inport
  Constant : Constant  Value=0
  Constant1 : Constant
  Demux : Demux  Outputs=9
  Multiport Switch : MultiPortSwitch  DataPortOrder=Zero-based contiguous  Inputs=11  zeroidx=on  SaturateOnIntegerOverflow=off  InputSameDT=off
  Pulse Generator : DiscretePulseGenerator  PulseType=Time based  Period=0.01  PulseWidth=[1 2 3 4 5 6 7 8 9]*10
  vSig : Outport  VectorParamsAs1DForOutWhenUnconnected=off
  wires:
  Multiport Switch/1 -> vSig/1
  Demux/9 -> Multiport Switch/11
  Demux/8 -> Multiport Switch/10
  Demux/7 -> Multiport Switch/9
  Demux/6 -> Multiport Switch/8
  Demux/5 -> Multiport Switch/7
  Demux/4 -> Multiport Switch/6
  Demux/3 -> Multiport Switch/5
  Demux/2 -> Multiport Switch/4
  Demux/1 -> Multiport Switch/3
  OnT/1 -> Multiport Switch/1
  Constant1/1 -> Multiport Switch/12
  Constant/1 -> Multiport Switch/2
  Pulse Generator/1 -> Demux/1

== system sm_car_/Controller/TrqVec 4Motor/Brake Control/ABS/Valve Control R2/Subsystem1 ==
  OnT : Inport
  Constant : Constant  Value=0
  Constant1 : Constant
  Demux : Demux  Outputs=9
  Multiport Switch : MultiPortSwitch  DataPortOrder=Zero-based contiguous  Inputs=11  zeroidx=on  SaturateOnIntegerOverflow=off  InputSameDT=off
  Pulse Generator : DiscretePulseGenerator  PulseType=Time based  Period=0.01  PulseWidth=[1 2 3 4 5 6 7 8 9]*10
  vSig : Outport  VectorParamsAs1DForOutWhenUnconnected=off
  wires:
  Pulse Generator/1 -> Demux/1
  Constant/1 -> Multiport Switch/2
  Constant1/1 -> Multiport Switch/12
  OnT/1 -> Multiport Switch/1
  Demux/1 -> Multiport Switch/3
  Demux/2 -> Multiport Switch/4
  Demux/3 -> Multiport Switch/5
  Demux/4 -> Multiport Switch/6
  Demux/5 -> Multiport Switch/7
  Demux/6 -> Multiport Switch/8
  Demux/7 -> Multiport Switch/9
  Demux/8 -> Multiport Switch/10
  Demux/9 -> Multiport Switch/11
  Multiport Switch/1 -> vSig/1

== system sm_car_/Controller/TrqVec_FLC_V3/Power Control/State Estimation/Sensor Noise Simulation/noise a_x ==
  <w> : Inport
  Add2 : Sum
  Band-Limited White Noise2 : simulink/Sources/Band-Limited White Noise  Cov=[1.22e-4]  Ts=0.01  seed=[512361]
  Quantizer2 : Quantizer  QuantizationInterval=0.0047
  Zero-Order Hold2 : ZeroOrderHold  SampleTime=0.01
  a_x_n : Outport
  wires:
  Quantizer2/1 -> Zero-Order Hold2/1
  Band-Limited White Noise2/1 -> Add2/2
  Zero-Order Hold2/1 -> Add2/1
  <w>/1 -> Quantizer2/1
  Add2/1 -> a_x_n/1  "a_x_n"

== system sm_car_/Controller/TrqVec_FLC_V3/Power Control/State Estimation/Sensor Noise Simulation/noise a_y ==
  <w> : Inport
  Add2 : Sum
  Band-Limited White Noise2 : simulink/Sources/Band-Limited White Noise  Cov=[1.22e-4]  Ts=0.01  seed=[092756]
  Quantizer2 : Quantizer  QuantizationInterval=0.0047
  Zero-Order Hold2 : ZeroOrderHold  SampleTime=0.01
  a_y_n : Outport
  wires:
  Quantizer2/1 -> Zero-Order Hold2/1
  Band-Limited White Noise2/1 -> Add2/2
  Zero-Order Hold2/1 -> Add2/1
  <w>/1 -> Quantizer2/1
  Add2/1 -> a_y_n/1  "a_y_n"

== system sm_car_/Controller/TrqVec_FLC_V3/Power Control/State Estimation/Sensor Noise Simulation/noise omega_fl ==
  <w> : Inport
  Add2 : Sum
  Band-Limited White Noise2 : simulink/Sources/Band-Limited White Noise  Cov=[1e-4]  Ts=0.01  seed=[12451]
  Quantizer2 : Quantizer  QuantizationInterval=2 * pi / 25
  Zero-Order Hold2 : ZeroOrderHold  SampleTime=0.01
  omega_rl : Outport
  wires:
  Quantizer2/1 -> Zero-Order Hold2/1
  Band-Limited White Noise2/1 -> Add2/2
  Zero-Order Hold2/1 -> Add2/1
  <w>/1 -> Quantizer2/1
  Add2/1 -> omega_rl/1  "omega_rl"

== system sm_car_/Controller/TrqVec_FLC_V3/Power Control/State Estimation/Sensor Noise Simulation/noise omega_fr ==
  <w> : Inport
  Add3 : Sum
  Band-Limited White Noise3 : simulink/Sources/Band-Limited White Noise  Cov=[1e-4]  Ts=0.01  seed=[68595]
  Quantizer3 : Quantizer  QuantizationInterval=2 * pi / 25
  Zero-Order Hold3 : ZeroOrderHold  SampleTime=0.01
  omega_rr : Outport
  wires:
  Quantizer3/1 -> Zero-Order Hold3/1
  <w>/1 -> Quantizer3/1
  Zero-Order Hold3/1 -> Add3/1
  Band-Limited White Noise3/1 -> Add3/2
  Add3/1 -> omega_rr/1  "omega_rr"

== system sm_car_/Controller/TrqVec_FLC_V3/Power Control/State Estimation/Sensor Noise Simulation/noise omega_rl ==
  <w> : Inport
  Add : Sum
  Band-Limited White Noise : simulink/Sources/Band-Limited White Noise  Cov=[1e-4]  Ts=0.01  seed=[23341]
  Quantizer : Quantizer  QuantizationInterval=2 * pi / 94
  Zero-Order Hold : ZeroOrderHold  SampleTime=0.01
  omega_rl : Outport
  wires:
  Zero-Order Hold/1 -> Add/1
  Add/1 -> omega_rl/1  "omega_rl"
  Band-Limited White Noise/1 -> Add/2
  <w>/1 -> Quantizer/1
  Quantizer/1 -> Zero-Order Hold/1

== system sm_car_/Controller/TrqVec_FLC_V3/Power Control/State Estimation/Sensor Noise Simulation/noise omega_rr ==
  <w> : Inport
  Add1 : Sum
  Band-Limited White Noise1 : simulink/Sources/Band-Limited White Noise  Cov=[1e-4]  Ts=0.01  seed=[41245]
  Quantizer1 : Quantizer  QuantizationInterval=2 * pi / 94
  Zero-Order Hold1 : ZeroOrderHold  SampleTime=0.01
  omega_rr : Outport
  wires:
  Zero-Order Hold1/1 -> Add1/1
  Band-Limited White Noise1/1 -> Add1/2
  <w>/1 -> Quantizer1/1
  Quantizer1/1 -> Zero-Order Hold1/1
  Add1/1 -> omega_rr/1  "omega_rr"

== system sm_car_/Controller/TrqVec_FLC_V3/Power Control/State Estimation/Sensor Noise Simulation/noise v_gps ==
  <vx> : Inport
  <vy> : Inport  Port=2
  <vz> : Inport  Port=3
  Add : Sum  Inputs=+++
  Add2 : Sum
  Band-Limited White Noise2 : simulink/Sources/Band-Limited White Noise  Cov=[9e-4]  Ts=0.1  seed=[645743]
  Quantizer2 : Quantizer  QuantizationInterval=0.01
  Sqrt : Sqrt
  Square : Math  Operator=square
  Square1 : Math  Operator=square
  Square2 : Math  Operator=square
  Zero-Order Hold2 : ZeroOrderHold  SampleTime=0.1
  V_n : Outport
  wires:
  Sqrt/1 -> Quantizer2/1
  Add/1 -> Sqrt/1
  Square2/1 -> Add/3
  Square1/1 -> Add/2
  <vz>/1 -> Square2/1
  <vy>/1 -> Square1/1
  Square/1 -> Add/1
  Add2/1 -> V_n/1  "V_n"
  <vx>/1 -> Square/1
  Zero-Order Hold2/1 -> Add2/1
  Band-Limited White Noise2/1 -> Add2/2
  Quantizer2/1 -> Zero-Order Hold2/1

== system sm_car_/Controller/TrqVec_FLC_V3/Power Control/State Estimation/Sensor Noise Simulation/noise yaw rate ==
  <w> : Inport
  Add2 : Sum
  Band-Limited White Noise2 : simulink/Sources/Band-Limited White Noise  Cov=[7.29e-7]  Ts=0.01  seed=[809953]
  Quantizer2 : Quantizer  QuantizationInterval=0.001
  Zero-Order Hold2 : ZeroOrderHold  SampleTime=0.01
  nYaw_n : Outport
  wires:
  Add2/1 -> nYaw_n/1  "nYaw_n"
  <w>/1 -> Quantizer2/1
  Zero-Order Hold2/1 -> Add2/1
  Band-Limited White Noise2/1 -> Add2/2
  Quantizer2/1 -> Zero-Order Hold2/1

== system sm_car_/Driver/Closed Loop/Maneuver/PoseTargetVisual/Count Lap/Triggered Subsystem ==
  Up Down : Inport
  Trigger : TriggerPort  VariantControl=Variant  ZeroCross=off
  Memory : Memory  InheritSampleTime=on
  Sum : Sum  Inputs=|++
  Num Laps : Outport  VectorParamsAs1DForOutWhenUnconnected=off
  wires:
  Up Down/1 -> Sum/2
  Sum/1 -> Num Laps/1, Memory/1
  Memory/1 -> Sum/1

== system sm_car_/Vehicle/Vehicle/Chassis/Aero/Subsystem/Actuator dynamics ==
  In : Inport
  Gain : Gain  Gain=1/b
  Integrator : Integrator  InitialCondition=x_initial*b
  Sum : Sum  Inputs=|+-  InputSameDT=on  SaturateOnIntegerOverflow=on  OutDataTypeStr=Inherit: Same as first input
  Out : Outport  VectorParamsAs1DForOutWhenUnconnected=off
  wires:
  Sum/1 -> Integrator/1
  In/1 -> Sum/1
  Integrator/1 -> Gain/1
  Gain/1 -> Sum/2, Out/1

== system sm_car_/Vehicle/Vehicle/Chassis/Body/Body Geometry/CAD FSAE Achilles ==
  Aero : Subsystem
  Body : Subsystem
  Rollbar : sm_lib/Body Elements/File Solid  ExtGeomFileName=FSAE_Rollbar.STL  UnitType=Custom  ExtGeomFileUnits=m  StepReaderType=HEX  ExportConvexHullGeometry=off  InertiaType=PointMass  BasedOnType=Density  Density=700.769  DensityUnits=kg/m^3  Mass=0  MassUnits=kg  CenterOfMass=[0.988684, 1.00464/1.8, 2.92072]  CenterOfMassUnits=m  MomentsOfInertia=[478.463, 518.088, 108.52]  MomentsOfInertiaUnits=kg*m^2  ProductsOfInertia=[-18.6469, 0.0347848, 0.00267861]  ProductsOfInertiaUnits=kg*m^2  GraphicType=FromGeometry  MarkerShape=Sphere  MarkerSize=10  GraphicVisPropType=SimpleVisualProperties  GraphicDiffuseColor=[0.6 0.6 0.6]  GraphicOpacity=1  GraphicSpecularColor=[0.5 0.5 0.5 1.0]  GraphicAmbientColor=[0.15 0.15 0.15 1.0]  GraphicEmissiveColor=[0.0 0.0 0.0 1.0]  GraphicShininess=75  DoExposeReferenceFrame=on  SerializedFrames=<Frames/>
  Seat : sm_lib/Body Elements/File Solid  ExtGeomFileName=FSAE_Seat.STL  UnitType=Custom  ExtGeomFileUnits=m  StepReaderType=HEX  ExportConvexHullGeometry=off  InertiaType=PointMass  BasedOnType=Density  Density=700.769  DensityUnits=kg/m^3  Mass=0  MassUnits=kg  CenterOfMass=[0.988684, 1.00464/1.8, 2.92072]  CenterOfMassUnits=m  MomentsOfInertia=[478.463, 518.088, 108.52]  MomentsOfInertiaUnits=kg*m^2  ProductsOfInertia=[-18.6469, 0.0347848, 0.00267861]  ProductsOfInertiaUnits=kg*m^2  GraphicType=FromGeometry  MarkerShape=Sphere  MarkerSize=10  GraphicVisPropType=SimpleVisualProperties  GraphicDiffuseColor=[0.2 0.2 0.2]  GraphicOpacity=1  GraphicSpecularColor=[0.5 0.5 0.5 1.0]  GraphicAmbientColor=[0.15 0.15 0.15 1.0]  GraphicEmissiveColor=[0.0 0.0 0.0 1.0]  GraphicShininess=75  DoExposeReferenceFrame=on  SerializedFrames=<Frames/>
  Transform CAD Offset : sm_lib/Frames and Transforms/Rigid Transform  RotationMethod=RotationSequence  FollAlignAxisA=+Y  BaseAlignAxisA=+Z  FollAlignAxisB=-X  BaseAlignAxisB=+Y  RotationStandardAxis=+Z  RotationAngle=0  RotationAngleUnits=deg  RotationArbitraryAxis=[0 0 1]  RotationSequenceAxes=FollowerAxes  RotationSequence=ZYX  RotationSequenceAngles=[body_orient(3) body_orient(2) body_orient(1)]  RotationSequenceAnglesUnits=rad  RotationMatrix=[1 0 0; 0 1 0; 0 0 1]  Quaternion=[1 0 0 0]  TranslationMethod=Cartesian  TranslationCartesianOffset=body_offset  TranslationCartesianOffsetUnits=m  TranslationStandardAxis=+Z  TranslationStandardOffset=0  TranslationStandardOffsetUnits=m  TranslationROffset=0  TranslationROffsetUnits=m  TranslationThetaOffset=0  TranslationThetaOffsetUnits=deg  TranslationZOffset=0  TranslationZOffsetUnits=m
  FA : PMIOPort  Side=Right
  P : PMIOPort  Port=2  Side=Left
  connections:
  Aero/RConn1 -- Transform CAD Offset/RConn1 -- Seat/RConn1 -- Body/LConn1 -- Rollbar/RConn1
  FA/RConn1 -- P/RConn1 -- Transform CAD Offset/LConn1

== system sm_car_/Vehicle/Vehicle/Chassis/Body/Body Load/None ==
  FA : PMIOPort  Side=Left

== system sm_car_/Vehicle/Vehicle/Chassis/Body/Body Sensor/Roll Pitch ==
  R : Inport
  Atan1 : Trigonometry  Operator=atan2
  Calculate aPitch : Subsystem
  Calculate aRoll : Subsystem
  Demux1 : Demux  Outputs=2
  "Flip sign for -x axis " : Gain  Gain=-1
  "R([2 1], 1)" : Selector  NumberOfDimensions=2  InputPortWidth=3  IndexOptions=Index vector (dialog),Index vector (dialog)  Indices=[2 1],1  OutputSizes=1,1  RuntimeRangeChecks=off
  Reshape : Reshape
  Select x axis : Selector  NumberOfDimensions=2  InputPortWidth=2  IndexOptions=Index vector (dialog),Index vector (dialog)  Indices=[1 2 3],1  OutputSizes=1,1  RuntimeRangeChecks=off
  Select y axis : Selector  NumberOfDimensions=2  InputPortWidth=2  IndexOptions=Index vector (dialog),Index vector (dialog)  Indices=[1 2 3],2  OutputSizes=1,1  RuntimeRangeChecks=off
  Transfer Fcn : TransferFcn  Numerator=[1 0]  Denominator=[0.01 1]
  Transfer Fcn1 : TransferFcn  Numerator=[1 0]  Denominator=[0.01 1]
  aRoll : Outport  VectorParamsAs1DForOutWhenUnconnected=off
  aPitch : Outport  Port=2  VectorParamsAs1DForOutWhenUnconnected=off
  nRoll : Outport  Port=3  VectorParamsAs1DForOutWhenUnconnected=off
  nPitch : Outport  Port=4  VectorParamsAs1DForOutWhenUnconnected=off
  aYaw : Outport  Port=5  VectorParamsAs1DForOutWhenUnconnected=off
  wires:
  Calculate aPitch/1(Angle) -> "Flip sign for -x axis "/1
  Select x axis/1 -> Calculate aPitch/2(uvec)
  Select y axis/1 -> Calculate aRoll/1(uvec)
  "Flip sign for -x axis "/1 -> aPitch/1, Transfer Fcn1/1
  Calculate aRoll/1(Angle) -> Transfer Fcn/1, aRoll/1, Calculate aPitch/1(Roll Angle)
  Transfer Fcn/1 -> nRoll/1
  Transfer Fcn1/1 -> nPitch/1
  Demux1/2 -> Atan1/2
  Atan1/1 -> Reshape/1
  "R([2 1], 1)"/1 -> Demux1/1
  Reshape/1 -> aYaw/1
  Demux1/1 -> Atan1/1
  R/1 -> "R([2 1], 1)"/1, Select y axis/1, Select x axis/1

== system sm_car_/Vehicle/Vehicle/Chassis/Damper/Decoupled/Damper A1 Heave ==
  "Ctrl " : Inport
  Linear : Subsystem  VariantControl=Linear  mask(Linear Damper with Bumpstop){dam_b=Damper.Damping.d.Value, hp_dpr_top=Damper.Damping.sTop.Value, hp_dpr_bot=Damper.Damping.sBottom.Value, bs_lim_upper=Damper.Endstop.xMax.Value, bs_lim_lower=Damper.Endstop.xMin.Value, bs_k_upper=Damper.Endstop.KxMax.Value, bs_k_lower=Damper.Endstop.KxMin.Value, bs_b_upper=Damper.Endstop.dxMax.Value, bs_b_lower=Damper.Endstop.dxMin.Value, bs_region=Damper.Endstop.xTransition.Value}
      mask prompts: dam_b "Damper (N/(m/s))"; hp_dpr_top "HP Damper Top [xyz] (m)"; hp_dpr_bot "HP Damper Bottom [xyz] (m)"; bs_region "Transition Region (m)"
      mask help: Linear damper with bumpstop at top and bottom.
      mask init:
      | dam_x0 = norm(hp_dpr_top - hp_dpr_bot);
      mask TypeOptions dam_b: Damper/D
      mask DialogControl text_bumpstop_upper Prompt: Upper
      mask DialogControl text_bumpstop_lower Prompt: Lower
      mask DialogControl text_bumpstop_limit Prompt: Limit (m)
      mask DialogControl text_bumpstop_k Prompt: Stiffness (N/m)
      mask DialogControl text_bumpstop_b Prompt: Damping  (N/(m/s))
  Nonlinear : Subsystem  VariantControl=Nonlinear  mask(Nonlinear Damper with Bumpstop){velocity_vector=Damper.Damping.vDamper.Value, force_vector=Damper.Damping.fDamper.Value, hp_dpr_top=Damper.Damping.sTop.Value, hp_dpr_bot=Damper.Damping.sBottom.Value, bs_lim_upper=Damper.Endstop.xMax.Value, bs_lim_lower=Damper.Endstop.xMin.Value, bs_k_upper=Damper.Endstop.KxMax.Value, bs_k_lower=Damper.Endstop.KxMin.Value, bs_b_upper=Damper.Endstop.dxMax.Value, bs_b_lower=Damper.Endstop.dxMin.Value, bs_region=Damper.Endstop.xTransition.Value}
      mask prompts: velocity_vector "Velocity vector"; force_vector "Force vector"; hp_dpr_top "HP Damper Top [xyz] (m)"; hp_dpr_bot "HP Damper Bottom [xyz] (m)"; bs_region "Transition Region (m)"
      mask help: Damper with damping coefficient specified as a lookup table in parallel with a bumpstop.
      mask init:
      | dam_x0 = norm(hp_dpr_top - hp_dpr_bot);
      mask TypeOptions velocity_vector: Damper/velocity_vector
      mask TypeOptions force_vector: Damper/force_vector
      mask DialogControl text_bumpstop_upper Prompt: Upper
      mask DialogControl text_bumpstop_lower Prompt: Lower
      mask DialogControl text_bumpstop_limit Prompt: Limit (m)
      mask DialogControl text_bumpstop_k Prompt: Stiffness (N/m)
      mask DialogControl text_bumpstop_b Prompt: Damping  (N/(m/s))
  " R" : PMIOPort  Side=Left
  " C" : PMIOPort  Port=2  Side=Right
  " meas" : Outport  VectorParamsAs1DForOutWhenUnconnected=off

== system sm_car_/Vehicle/Vehicle/Chassis/Damper/Decoupled/Damper A1 Roll ==
  "Ctrl " : Inport
  Linear : Subsystem  VariantControl=Linear  mask(Linear Damper with Bumpstop){dam_b=Damper.Damping.d.Value, hp_dpr_top=Damper.Damping.sTop.Value, hp_dpr_bot=Damper.Damping.sBottom.Value, bs_lim_upper=Damper.Endstop.xMax.Value, bs_lim_lower=Damper.Endstop.xMin.Value, bs_k_upper=Damper.Endstop.KxMax.Value, bs_k_lower=Damper.Endstop.KxMin.Value, bs_b_upper=Damper.Endstop.dxMax.Value, bs_b_lower=Damper.Endstop.dxMin.Value, bs_region=Damper.Endstop.xTransition.Value}
      mask prompts: dam_b "Damper (N/(m/s))"; hp_dpr_top "HP Damper Top [xyz] (m)"; hp_dpr_bot "HP Damper Bottom [xyz] (m)"; bs_region "Transition Region (m)"
      mask help: Linear damper with bumpstop at top and bottom.
      mask init:
      | dam_x0 = norm(hp_dpr_top - hp_dpr_bot);
      mask TypeOptions dam_b: Damper/D
      mask DialogControl text_bumpstop_upper Prompt: Upper
      mask DialogControl text_bumpstop_lower Prompt: Lower
      mask DialogControl text_bumpstop_limit Prompt: Limit (m)
      mask DialogControl text_bumpstop_k Prompt: Stiffness (N/m)
      mask DialogControl text_bumpstop_b Prompt: Damping  (N/(m/s))
  Nonlinear : Subsystem  VariantControl=Nonlinear  mask(Nonlinear Damper with Bumpstop){velocity_vector=Damper.Damping.vDamper.Value, force_vector=Damper.Damping.fDamper.Value, hp_dpr_top=Damper.Damping.sTop.Value, hp_dpr_bot=Damper.Damping.sBottom.Value, bs_lim_upper=Damper.Endstop.xMax.Value, bs_lim_lower=Damper.Endstop.xMin.Value, bs_k_upper=Damper.Endstop.KxMax.Value, bs_k_lower=Damper.Endstop.KxMin.Value, bs_b_upper=Damper.Endstop.dxMax.Value, bs_b_lower=Damper.Endstop.dxMin.Value, bs_region=Damper.Endstop.xTransition.Value}
      mask prompts: velocity_vector "Velocity vector"; force_vector "Force vector"; hp_dpr_top "HP Damper Top [xyz] (m)"; hp_dpr_bot "HP Damper Bottom [xyz] (m)"; bs_region "Transition Region (m)"
      mask help: Damper with damping coefficient specified as a lookup table in parallel with a bumpstop.
      mask init:
      | dam_x0 = norm(hp_dpr_top - hp_dpr_bot);
      mask TypeOptions velocity_vector: Damper/velocity_vector
      mask TypeOptions force_vector: Damper/force_vector
      mask DialogControl text_bumpstop_upper Prompt: Upper
      mask DialogControl text_bumpstop_lower Prompt: Lower
      mask DialogControl text_bumpstop_limit Prompt: Limit (m)
      mask DialogControl text_bumpstop_k Prompt: Stiffness (N/m)
      mask DialogControl text_bumpstop_b Prompt: Damping  (N/(m/s))
  " R" : PMIOPort  Side=Left
  " C" : PMIOPort  Port=2  Side=Right
  " meas" : Outport  VectorParamsAs1DForOutWhenUnconnected=off
